simulink model "EV6_LUT_FourWheel_EV6Battery77p4kWh_PowerCorrected"  (R2024a)
settings: Solver=ode4  StartTime=0  StopTime=60  FixedStep=0.001  RelTol=1e-3
PreLoadFcn:
  | VSS_BICYCLE=Simulink.Variant('Dual=0');
  | VSS_DUAL=Simulink.Variant('Dual=1');
  | Dual=1;
  | load('DriveCycle2.mat')
PostLoadFcn:
  | if any(exist('dsrtsu_mdlpostloadfcn', 'file') ~= 0), dsrtsu_mdlpostloadfcn('Execute', bdroot); end
InitFcn:
  | , if any(exist('rtifpga_mdlclblib', 'file') ~= 0), rtifpga_mdlclblib('Init', bdroot); end,
  | , if any(exist('dsmpb_private', 'file') ~= 0), dsmpb_private('dsmpb_mdlclblib', 'Init', bdroot); end,
  | load('DriveCycle2.mat')
model workspace (MAT data in the model file):
  DiffRatio = 10.65
  EV6_2023_BattBranchCapacity_Ah = 55.5236728838
  EV6_2023_BattEnergy_kWh = 77.4
  EV6_2023_BattNominalVoltage_V = 697
  EV6_2023_BattNumCellsParallel = 2
  EV6_2023_BattNumCellsSeries = 192
  EV6_2023_BattOpenVoltCapBpts = [0 0.1 0.2 0.3 0.4 0.5 0.6 0.7 0.8 0.9 1]
  EV6_2023_BattOpenVoltTbl = [2.96762142548 3.40364281191 3.47417488548 3.54470541822 3.61523441014 3.68576186124 3.75628777151 3.82681214095 3.94527005036 4.07101207308 4.2120755254]
  EV6_2023_BattPackCapacity_Ah = 111.047345768
  EV6_2023_BattResistSocBpts = [0 0.2 0.4 0.6 0.8 1]
  EV6_2023_BattResistTbl = [0.0163620057716 0.0118174152018 0.00807187352333 0.00375663957972 0.00266904525531 0.00103635901355 0.0019014404175 0.0172368903217 0.0121226074867 0.00758541551769 0.00474065349228 0.00337561163613 ... (42 elements, 7x6)]
  EV6_2023_BattResistTempBpts = [243.1 253.1 263.1 273.1 283.1 298.1 313.1]
  EV6_2023_InitialPackOCV_V = 726.471714233
  EV6_2023_InitialSOC = 0.638878863672
  EV6_BattCellCapacity_Ah = 60.3
  EV6_BattInitialSOC = 0.638878863672
  EV6_BattOCV_Cell_V = [2.96762142548 3.40364281191 3.47417488548 3.54470541822 3.61523441014 3.68576186124 3.75628777151 3.82681214095 3.94527005036 4.07101207308 4.2120755254]
  EV6_BattOCV_SOC = [0 0.1 0.2 0.3 0.4 0.5 0.6 0.7 0.8 0.9 1]
  EV6_BattPackCapacity_Ah = 120.6
  EV6_BattParallelCells = 2
  EV6_BattResistanceSOC = [0 0.2 0.4 0.6 0.8 1]
  EV6_BattResistanceTable_Ohm = [0.0163620057716 0.0118174152018 0.00807187352333 0.00375663957972 0.00266904525531 0.00103635901355 0.0019014404175 0.0172368903217 0.0121226074867 0.00758541551769 0.00474065349228 0.00337561163613 ... (42 elements, 7x6)]
  EV6_BattResistanceTemp_K = [243.1 253.1 263.1 273.1 283.1 298.1 313.1]
  EV6_BattSeriesCells = 192
  EV6_FinalDriveRatio = 10.65
  EV6_TargetPackResistance_Ohm = 0.132763804608
  Gas = 0.383333333333
undefined symbols (not defined in the file): accel_bp_mps2, AccelCmd, ActTqLF_Nm_, ActTqLR_Nm_, ActTqRF_Nm_, ActTqRR_Nm_, BattChargeLimitMaxPwr, BattChargeLimitSocBpts, BattChargeLimitTbl, BattDischargeLimitSocBpts, BattDischargeLimitTbl, BattDischargeMaxPwr, BrakeMaxPrs, BrakeMaxTrq, ChassisDistCg2FrontAxle, ChassisDistCg2RearAxle, ChassisVehMass, CltchCmd, CoastDown, DecelCmd, DiscIntNeverNeededParam, EnvGravCnst, EnvPrs, EnvTemp, EV6_RegenTorqueGain, EV6_TractionTorqueGain, front_share_regen_3d, front_share_traction_3d, FuelSpecificGrav, GearCmd, h, InitStates, lgSw, limitedMCT, MCT, MtrEffSpdBpts, MtrEffTbl, MtrEffTrqBpts, MtrPwrMax, MtrTrqMax, out_1, pMCT, RealSimPara, Ref_speed, Ref_time, regen_torque_bp_Nm, speed_bp_kph, SteeringCmd, SupvsryCtrlRegenBrkCutOffTbl, SupvsryCtrlRegenSpdBpts, TestScnrioCycleNum, traction_torque_bp_Nm, US06, VEH
libraries: VSIGenLib x65, simulink x54, etargetslib x38, dsmpblib x24, vehdynlibtire x12, autolibshared x11, vehdynlibsuspension x7, vehdynlibtirecommon x7, autolibpowerinfoutils x6, autolibutils x5, autolibsharedcoupling x4, autolibmappedmotor x4
(part 7 of 19)

== system EV6_LUT_FourWheel_EV6Battery77p4kWh_PowerCorrected/Vehicle Under Test1/Vehicle/Rototest and ORNL Interface/RotoTrqPreprocess ==
  AxleTrqRaw : Inport
  Bus Selector1 : BusSelector  OutputSignals=ActTqLF_Nm_,ActTqRF_Nm_,ActTqLR_Nm_,ActTqRR_Nm_
  Compare To Constant : simulink/Logic and Bit Operations/Compare To Constant  relop=>=  const=-15  OutDataTypeStr=boolean
  Compare To Constant1 : simulink/Logic and Bit Operations/Compare To Constant  relop=<=  const=0  OutDataTypeStr=boolean
  Data Type Conversion{1..4} (4 alike) : DataTypeConversion  OutDataTypeStr=double  SaturateOnIntegerOverflow=off  RndMeth=Floor
  FirstOrderFilterTau{,1..3} (4 alike) : VSIGenLib/FirstOrderFilterTau  SystemSampleTime=-1  VariantActivationTime=update diagram  AllowFlexibleInterface=on  Latency=0  AutoFrameSizeCalculation=off
  Ground : Ground
  Logical Operator : Logic  AllPortsSameDT=off  OutDataTypeStr=boolean
  ManualTrq_Nm : Constant  Value=0
  Mux : Mux
  Mux1 : Mux
  SatTrq : Saturate  UpperLimit=1000  LowerLimit=-1000
  Tau : Constant  Value=0.01
  TorqueIn : Switch  Criteria=u2 > Threshold  SaturateOnIntegerOverflow=off  InputSameDT=off
  "TorqueIn " : Switch  Criteria=u2 > Threshold  SaturateOnIntegerOverflow=off  InputSameDT=off
  AxleTrqRoto : Outport
  AxleTrqVeh : Outport  Port=2
  wires:
  Data Type Conversion1/1 -> Mux/1  "LF"
  FirstOrderFilterTau2/1 -> Data Type Conversion3/1
  SatTrq/1 -> Compare To Constant/1, Compare To Constant1/1, "TorqueIn "/3
  Compare To Constant1/1 -> Logical Operator/2
  Bus Selector1/1 -> FirstOrderFilterTau/1  "<ActTqLF_Nm_>"
  FirstOrderFilterTau3/1 -> Data Type Conversion4/1
  FirstOrderFilterTau/1 -> Data Type Conversion1/1
  AxleTrqRaw/1 -> Bus Selector1/1
  Data Type Conversion2/1 -> Mux/2  "RF"
  FirstOrderFilterTau1/1 -> Data Type Conversion2/1
  "TorqueIn "/1 -> AxleTrqVeh/1  "Trq"
  TorqueIn/1 -> SatTrq/1
  Bus Selector1/2 -> FirstOrderFilterTau1/1  "<ActTqRF_Nm_>"
  Bus Selector1/3 -> FirstOrderFilterTau2/1  "<ActTqLR_Nm_>"
  Compare To Constant/1 -> Logical Operator/1
  Bus Selector1/4 -> FirstOrderFilterTau3/1  "<ActTqRR_Nm_>"
  [Switch] -> TorqueIn/2
  Mux1/1 -> TorqueIn/3
  Data Type Conversion3/1 -> Mux/3  "LR"
  Data Type Conversion4/1 -> Mux/4  "RR"
  Logical Operator/1 -> "TorqueIn "/2
  Ground/1 -> "TorqueIn "/1
  Tau/1 -> FirstOrderFilterTau3/2, FirstOrderFilterTau2/2, FirstOrderFilterTau1/2, FirstOrderFilterTau/2
  ManualTrq_Nm/1 -> Mux1/1, Mux1/2, Mux1/3, Mux1/4
  Mux/1 -> TorqueIn/1, AxleTrqRoto/1

== system EV6_LUT_FourWheel_EV6Battery77p4kWh_PowerCorrected/Vehicle Under Test1/Vehicle/Rototest and ORNL Interface/Subsystem2 ==
  AxlTorq : Inport
  BusCreator1 : BusCreator  Inputs=16
  BusCreator2 : BusCreator  Inputs=16
  Constant : Constant  Value=0
  Constant1 : Constant  Value=0
  Demux : Demux  Outputs=16
      settings: DisplayOption=none
  Terminator : Terminator
  Zero1 : Constant  Value=0
  Zero2 : Constant  Value=0
  Zero5 : Constant  Value=0
  BrakeUpd : Outport
  wires:
  AxlTorq/1 -> Terminator/1
  Demux/12 -> BusCreator1/12  "Brake IF Trq_Reg_trg RR"
  Zero5/1 -> BusCreator2/5, BusCreator2/6, BusCreator2/7, BusCreator2/8  "Brake IF Trq_PB RR"
  Demux/7 -> BusCreator1/7  "Brake IF Trq_PB RL"
  Demux/5 -> BusCreator1/5  "Brake IF Trq_PB FL"
  Demux/13 -> BusCreator1/13  "Brake IF Trq_DriveSrc_trg d0"
  BusCreator2/1 -> Demux/1
  Demux/10 -> BusCreator1/10  "Brake IF Trq_Reg_trg FR"
  Demux/8 -> BusCreator1/8  "Brake IF Trq_PB RR"
  Demux/1 -> BusCreator1/1  "Brake IF Trq_WB FL"
  BusCreator1/1 -> BrakeUpd/1
  Constant/1 -> BusCreator2/3, BusCreator2/4  "Brake IF Trq_WB RL"
  Demux/3 -> BusCreator1/3  "Brake IF Trq_WB RL"
  Demux/4 -> BusCreator1/4  "Brake IF Trq_WB RR"
  Zero1/1 -> BusCreator2/9, BusCreator2/10, BusCreator2/11, BusCreator2/12  "Brake IF Trq_Reg_trg RR"
  Demux/16 -> BusCreator1/16  "Brake IF Trq_DriveSrc_trg d3"
  Demux/2 -> BusCreator1/2  "Brake IF Trq_WB FR"
  Demux/15 -> BusCreator1/15  "Brake IF Trq_DriveSrc_trg d2"
  Demux/11 -> BusCreator1/11  "Brake IF Trq_Reg_trg RL"
  Zero2/1 -> BusCreator2/13, BusCreator2/14, BusCreator2/15, BusCreator2/16  "Brake IF Trq_DriveSrc_trg d3"
  Demux/14 -> BusCreator1/14  "Brake IF Trq_DriveSrc_trg d1"
  Constant1/1 -> BusCreator2/2, BusCreator2/1  "Brake IF Trq_WB FL"
  Demux/6 -> BusCreator1/6  "Brake IF Trq_PB FR"
  Demux/9 -> BusCreator1/9  "Brake IF Trq_Reg_trg FL"

== system EV6_LUT_FourWheel_EV6Battery77p4kWh_PowerCorrected/Vehicle Under Test1/Vehicle/Rototest and ORNL Interface/To Rototest with Band-Aid ==
  note: Switch = 0 Overides
      | Switch = 1 Model
  note: OutMode = 0 is Torque
      | OutMode = 1 is Speed
  note: Torque Model: Low speed
      | Speed Model: Normal speed
  SpeedCmd_rps : Inport
  AxleTrq_roto_Nm : Inport  Port=2
  BRAKE_PRESSED : Inport  Port=3
  Vehicle_Speed_kph : Inport  Port=4
  Band-Aid : Subsystem
  Demux : Demux
  Demux1 : Demux
  Demux2 : Demux
  Logging : Subsystem  Commented=on
  MasterSw : Constant  Value=0
  Mode Override : Subsystem
  ModeOut : Switch  Criteria=u2 > Threshold  SaturateOnIntegerOverflow=off  InputSameDT=off
  ModeSwitch : MultiPortSwitch  DataPortOrder=Zero-based contiguous  Inputs=2  zeroidx=on  SaturateOnIntegerOverflow=off  InputSameDT=off
  Mux2 : Mux
  Mux4 : Mux
  Mux5 : Mux
  RateLimSpd : RateLimiter  RisingSlewLimit=500  FallingSlewLimit=-500  SampleTimeMode=inherited
  RotoTestEthTx : Subsystem  AncestorBlock=VSIGenLib/RotoTestEthTx
      mask Display:
      | color('white')
      | disp('RotTestEthTx')
      | port_label('input', 1, 'RefLF_NmORrpm')
      | port_label('input', 2, 'RefRF_NmORrpm')
      | port_label('input', 3, 'RefLR_NmORrpm')
      | port_label('input', 4, 'RefRR_NmORrpm')
      | port_label('input', 5, 'SqTrRR')
      | port_label('input', 6, 'SqTrLR')
      | port_label('input', 7, 'SqTrRF')
      | port_label('input', 8, 'SqTrLF')
      | port_label('input', 9, 'SystemActive')
      | port_label('output', 1, 'Status (bool)')
      | port_label('output', 2, 'Sent Bytes (int)')
  SatSpd : Saturate  UpperLimit=500  LowerLimit=0
  Scope : Scope
  SpeedOut : Switch  Criteria=u2 > Threshold  SaturateOnIntegerOverflow=off  InputSameDT=off
  SystemActive : Constant  Value=0  OutDataTypeStr=uint8
  Transfer Fcn{,1..3} (4 alike) : TransferFcn  Denominator=[0.02 1]
  TrqSpd Override : Subsystem
  ZeroTorque : Constant  Value=0  OutDataTypeStr=uint8
  rads2rpm : Gain  Gain=9.5492965964254
  Out1 : Outport
  tag scope: Switch=global
  wires:
  Transfer Fcn3/1 -> RotoTestEthTx/4(RefRR_NmORrpm)
  Transfer Fcn2/1 -> RotoTestEthTx/3(RefLR_NmORrpm)
  Transfer Fcn1/1 -> RotoTestEthTx/2(RefRF_NmORrpm)
  Transfer Fcn/1 -> RotoTestEthTx/1(RefLF_NmORrpm)
  Vehicle_Speed_kph/1 -> Band-Aid/4(VehSpd_kph)
  BRAKE_PRESSED/1 -> Band-Aid/3(BRAKE_PRESSED)
  Band-Aid/2(OutSpd_rpm) -> SpeedOut/1
  Mux2/1 -> Band-Aid/1(InSpd_rpm)
  AxleTrq_roto_Nm/1 -> Band-Aid/2(InTrq_Nm)
  Mode Override/1(Ovr) -> ModeOut/3
  SpeedCmd_rps/1 -> rads2rpm/1
  Demux2/4 -> RotoTestEthTx/8(SpTqLF)
  Demux1/2 -> Transfer Fcn1/1
  Demux1/1 -> Transfer Fcn/1
  RotoTestEthTx/1(Output) -> Out1/1  "ByteSend"
  SystemActive/1 -> RotoTestEthTx/9(SystemActive)
  Demux2/2 -> RotoTestEthTx/6(SpTqLR)
  Demux2/3 -> RotoTestEthTx/7(SpTqRF)
  Demux1/3 -> Transfer Fcn2/1
  Demux2/1 -> RotoTestEthTx/5(SpTqRR)
  Mux5/1 -> ModeOut/1
  [Switch] -> ModeOut/2
  SatSpd/1 -> ModeSwitch/3  "Spd"
  [Switch] -> SpeedOut/2
  ModeOut/1 -> Demux2/1
  Band-Aid/1(OutMode) -> ModeSwitch/1, Mux5/1, Mux5/2, Mux5/3, Mux5/4
  Demux/4 -> Mux2/4  "RRIn"
  ModeSwitch/1 -> Demux1/1, Scope/1
  rads2rpm/1 -> Demux/1
  RateLimSpd/1 -> SatSpd/1
  SpeedOut/1 -> RateLimSpd/1
  Demux/1 -> Mux2/1  "LFIn"
  ZeroTorque/1 -> Mux4/1, Mux4/4, Mux4/3, Mux4/2
  TrqSpd Override/1(Ovr) -> SpeedOut/3
  MasterSw/1 -> [Switch]
  Demux/2 -> Mux2/2  "RFIn"
  Demux1/4 -> Transfer Fcn3/1
  Demux/3 -> Mux2/3  "LRIn"
  Mux4/1 -> ModeSwitch/2

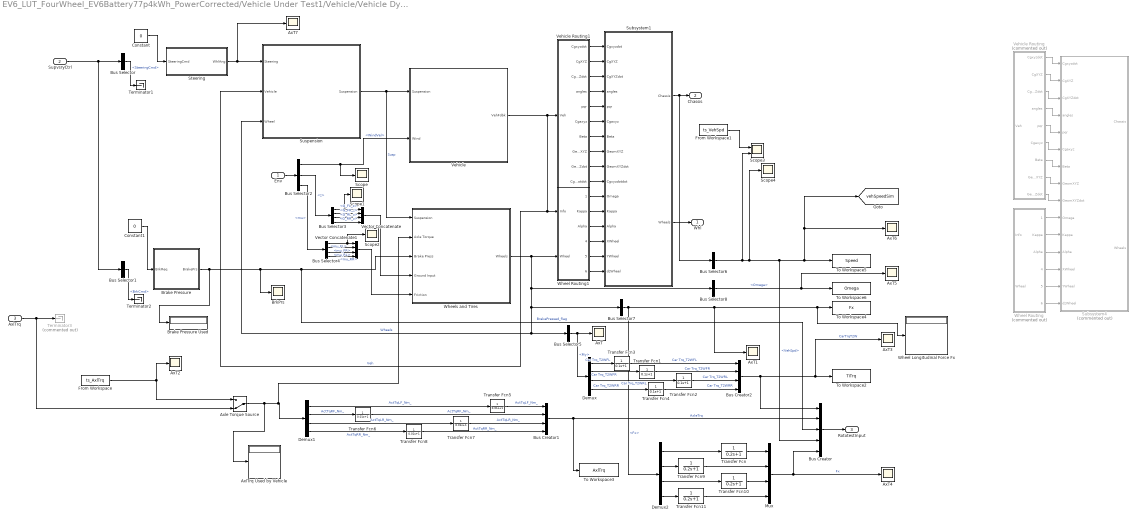
== system EV6_LUT_FourWheel_EV6Battery77p4kWh_PowerCorrected/Vehicle Under Test1/Vehicle/Vehicle Dynamics/Vehicle 14DOF ==
  Env : Inport
  SupvsryCtrl : Inport  Port=2
  AxlTrq : Inport  Port=3
  AxT{,1..7} (8 alike) : Scope
  AxlTrq Used by Vehicle : Display
  Axle Torque Source : ManualSwitch  CurrentSetting=0
  Brake Pressure : Subsystem
  Brake Pressure Used : Display
  BrkPrs : Scope
  Bus Creator : BusCreator  Inputs=5
  Bus Creator1 : BusCreator  Inputs=ActTqLF_Nm_,ActTqRF_Nm_,ActTqLR_Nm_,ActTqRR_Nm_
  Bus Creator2 : BusCreator  Inputs=Car Trq_T2WFL,Car Trq_T2WFR,Car Trq_T2WRL,Car Trq_T2WRR
  Bus Selector : BusSelector  OutputSignals=SteeringCmd
  Bus Selector1 : BusSelector  OutputSignals=BrkCmd
  Bus Selector2 : BusSelector  OutputSignals=WindVel,GndBus.z,GndBus.mu
  Bus Selector3 : BusSelector  OutputSignals=G_FL_z,G_FR_z,G_RL_z,G_RR_z
  Bus Selector4 : BusSelector  OutputSignals=mu_FL,mu_FR,mu_RL,mu_RR
  Bus Selector5 : BusSelector  OutputSignals=TireFrame.My
  Bus Selector6 : BusSelector  OutputSignals=VehSpd
  Bus Selector7 : BusSelector  OutputSignals=TireFrame.Fx
  Bus Selector8 : BusSelector  OutputSignals=TireFrame.Omega
  Constant : Constant  Value=0
  Constant1 : Constant  Value=0
  Demux : Demux
  Demux1 : Demux
  Demux2 : Demux
  From Workspace : FromWorkspace  VariableName=ts_AxlTrq
  From Workspace1 : FromWorkspace  VariableName=ts_VehSpd
  Mux : Mux
  Scope{,1..2,4} (4 alike) : Scope
  Scope3 : Scope  NumInputPorts=2
  Steering : Subsystem
  Subsystem1 : Subsystem
  Subsystem4 : Subsystem  Commented=on
  Suspension : Subsystem  Variant=on  VariantControlMode=label  LabelModeActiveChoice=3
      mask Display:
      | switch str2num(get_param(gcb,'ActiveVariant'))
      |     case 1
      |         image('suspdw.png');
      |     case 2
      |         image([imread('suspindmap.png');imread('suspsamap.png')]);
      |     case 3
      |          image([imread('suspmacp.png');imread('suspsacoil.png')]);
      |     case 4
      |          image('suspmacp.png');
      |     case 5
      |          image('suspindmap.png');
      | end
  Terminator1 : Terminator
  Terminator2 : Terminator
  Terminator3 : Terminator  Commented=on
  To Workspace2 : ToWorkspace  VariableName=TiTrq  SampleTime=-1
      settings: Save2DSignal=2-D array (concatenate along first dimension)
  To Workspace3 : ToWorkspace  VariableName=AxlTrq  SampleTime=-1
      settings: Save2DSignal=2-D array (concatenate along first dimension)
  To Workspace4 : ToWorkspace  VariableName=Fx  SampleTime=-1
      settings: Save2DSignal=2-D array (concatenate along first dimension)
  To Workspace5 : ToWorkspace  VariableName=Speed  SampleTime=-1
      settings: Save2DSignal=2-D array (concatenate along first dimension)
  To Workspace6 : ToWorkspace  VariableName=Omega  SampleTime=-1
      settings: Save2DSignal=2-D array (concatenate along first dimension)
  Transfer Fcn{,9..11} (4 alike) : TransferFcn  Denominator=[0.2 1]
  Transfer Fcn{1..4} (4 alike) : TransferFcn  Denominator=[0.1 1]
  Transfer Fcn{5..8} (4 alike) : TransferFcn  Denominator=[0.01 1]
  Vector Concatenate : Concatenate  NumInputs=4
  Vector Concatenate1 : Concatenate  NumInputs=4
  Vehicle : Subsystem
      mask Display: image('6dofcar.png');
  Vehicle Routing : Subsystem  Commented=on
  Vehicle Routing1 : Subsystem
  Wheel Longitudinal Force Fx : Display
  Wheel Routing : Subsystem  Commented=on
  Wheel Routing1 : Subsystem
  Wheels and Tires : Subsystem
      mask Display: image('wheel3dof.png')
  Whl : Outport
  Chassis : Outport  Port=2
  RototestInput : Outport  Port=3
  tag scope: vehSpeedSim=global
  wires:
  Vehicle Routing1/9(GeomXYZdot) -> Subsystem1/9(GeomXYZdot)
  Vehicle Routing1/8(GeomXYZ) -> Subsystem1/8(GeomXYZ)
  Vehicle Routing1/1(Cgxyzdot) -> Subsystem1/1(Cgxyzdot)
  Vehicle Routing1/5(pqr) -> Subsystem1/5(pqr)
  Vehicle Routing1/4(angles) -> Subsystem1/4(angles)
  Vehicle Routing1/3(CgXYZdot) -> Subsystem1/3(CgXYZdot)
  Vehicle Routing1/7(Beta) -> Subsystem1/7(Beta)
  Vehicle Routing1/2(CgXYZ) -> Subsystem1/2(CgXYZ)
  Vehicle Routing1/6(Cgaxyz) -> Subsystem1/6(Cgaxyz)
  Wheel Routing1/1(Omega) -> Subsystem1/11(Omega)
  Wheel Routing1/3(Alpha) -> Subsystem1/13(Alpha)
  Wheel Routing1/4(XWheel) -> Subsystem1/14(XWheel)
  Wheel Routing1/2(Kappa) -> Subsystem1/12(Kappa)
  Wheel Routing1/5(YWheel) -> Subsystem1/15(YWheel)
  Wheel Routing1/6(ZWheel) -> Subsystem1/16(dzWheel)
  Vehicle Routing1/10(Cgxyzdotdot) -> Subsystem1/10(Cgxyzdotdot)
  Vehicle Routing/8(GeomXYZ) -> Subsystem4/8(GeomXYZ)
  Vehicle Routing/6(Cgaxyz) -> Subsystem4/6(Cgaxyz)
  Vehicle Routing/3(CgXYZdot) -> Subsystem4/3(CgXYZdot)
  Vehicle Routing/9(GeomXYZdot) -> Subsystem4/9(GeomXYZdot)
  Vehicle Routing/4(angles) -> Subsystem4/4(angles)
  Vehicle Routing/7(Beta) -> Subsystem4/7(Beta)
  Wheel Routing/4(XWheel) -> Subsystem4/13(XWheel)
  Wheel Routing/1(Omega) -> Subsystem4/10(Omega)
  Wheel Routing/3(Alpha) -> Subsystem4/12(Alpha)
  Wheel Routing/5(YWheel) -> Subsystem4/14(YWheel)
  Wheel Routing/6(ZWheel) -> Subsystem4/15(dzWheel)
  Wheel Routing/2(Kappa) -> Subsystem4/11(Kappa)
  Vehicle Routing/1(Cgxyzdot) -> Subsystem4/1(Cgxyzdot)
  Vehicle Routing/5(pqr) -> Subsystem4/5(pqr)
  Vehicle Routing/2(CgXYZ) -> Subsystem4/2(CgXYZ)
  Transfer Fcn2/1 -> Bus Creator2/3  "Car Trq_T2WRL"
  Transfer Fcn4/1 -> Bus Creator2/4  "Car Trq_T2WRR"
  Demux/4 -> Transfer Fcn4/1  "Car Trq_T2WRR"
  Demux/1 -> Transfer Fcn3/1  "Car Trq_T2WFL"
  Demux/2 -> Transfer Fcn1/1  "Car Trq_T2WFR"
  Transfer Fcn1/1 -> Bus Creator2/2  "Car Trq_T2WFR"
  Demux/3 -> Transfer Fcn2/1  "Car Trq_T2WRL"
  Transfer Fcn3/1 -> Bus Creator2/1  "Car Trq_T2WFL"
  Mux/1 -> AxT4/1, Bus Creator/5  "Fx"
  Transfer Fcn11/1 -> Mux/4
  Demux2/1 -> Transfer Fcn/1
  Transfer Fcn/1 -> Mux/1
  Demux2/4 -> Transfer Fcn11/1
  Transfer Fcn9/1 -> Mux/2
  Demux2/2 -> Transfer Fcn9/1
  Transfer Fcn10/1 -> Mux/3
  Demux2/3 -> Transfer Fcn10/1
  Demux1/4 -> Transfer Fcn8/1  "ActTqRR_Nm_"
  Transfer Fcn7/1 -> Bus Creator1/3  "ActTqLR_Nm_"
  Demux1/1 -> Transfer Fcn5/1  "ActTqLF_Nm_"
  Transfer Fcn6/1 -> Bus Creator1/2  "ActTqRF_Nm_"
  Demux1/2 -> Transfer Fcn6/1  "ActTqRF_Nm_"
  Transfer Fcn8/1 -> Bus Creator1/4  "ActTqRR_Nm_"
  Demux1/3 -> Transfer Fcn7/1  "ActTqLR_Nm_"
  Transfer Fcn5/1 -> Bus Creator1/1  "ActTqLF_Nm_"
  Bus Creator/1 -> RototestInput/1
  Bus Selector8/1 -> To Workspace6/1, AxT5/1  "<Omega>"
  Bus Selector7/1 -> Wheel Longitudinal Force Fx/1, To Workspace4/1, AxT1/1, Demux2/1  "<Fx>"
  Subsystem1/1(Chassis) -> Chassis/1, Bus Selector6/1
  Bus Selector5/1 -> AxT/1, Demux/1  "<My>"
  Bus Creator2/1 -> To Workspace2/1, AxT3/1, Bus Creator/1  "CarTrqT2W"
  Bus Creator1/1 -> Bus Creator/2, To Workspace3/1  "AxleTrq"
  Brake Pressure/1(BrakePrs) -> Brake Pressure Used/1, Wheels and Tires/3(Brake Press), Bus Creator/3, BrkPrs/1  "BrakePressed_flag"
  Bus Selector6/1 -> Scope3/2, Scope4/1, Bus Creator/4, To Workspace5/1, [vehSpeedSim], AxT6/1  "<VehSpd>"
  Vector Concatenate1/1 -> Wheels and Tires/5(Friction)
  Bus Selector4/1 -> Vector Concatenate1/1, Scope2/1  "<mu_FL>"
  Bus Selector4/2 -> Vector Concatenate1/2  "<mu_FR>"
  Bus Selector4/3 -> Vector Concatenate1/3  "<mu_RL>"
  Bus Selector2/3 -> Bus Selector4/1  "<mu>"
  Bus Selector4/4 -> Vector Concatenate1/4  "<mu_RR>"
  Vector Concatenate/1 -> Wheels and Tires/4(Ground Input)
  Bus Selector3/4 -> Vector Concatenate/4  "<G_RR_z>"
  Bus Selector3/3 -> Vector Concatenate/3  "<G_RL_z>"
  Bus Selector3/2 -> Vector Concatenate/2  "<G_FR_z>"
  Bus Selector3/1 -> Vector Concatenate/1, Scope1/1  "<G_FL_z>"
  Bus Selector2/2 -> Bus Selector3/1  "<z>"
  Subsystem1/2(Wheels) -> Whl/1
  Env/1 -> Bus Selector2/1
  SupvsryCtrl/1 -> Bus Selector1/1, Bus Selector/1
  Steering/1(WhlAng) -> Suspension/1(Steering), AxT7/1
  Bus Selector2/1 -> Vehicle/2(Wind), Scope/1  "<WindVel>"
  Suspension/1(Suspension) -> Wheels and Tires/1(Suspension), Vehicle/1(Suspension)  "Susp"
  Vehicle/1(VehFdbk) -> Suspension/2(Vehicle), Wheel Routing1/1(Info), Vehicle Routing1/1(Veh)  "Veh"
  Wheels and Tires/1(Wheels) -> Wheel Routing1/2(Wheel), Bus Selector8/1, Suspension/3(Wheel), Bus Selector5/1, Bus Selector7/1  "Wheels"
  From Workspace1/1 -> Scope3/1
  From Workspace/1 -> Axle Torque Source/1, AxT2/1
  AxlTrq/1 -> Axle Torque Source/2, Terminator3/1
  Bus Selector1/1 -> Terminator2/1  "<BrkCmd>"
  Constant1/1 -> Brake Pressure/1(BrkReq)
  Constant/1 -> Steering/1(SteeringCmd)
  Bus Selector/1 -> Terminator1/1  "<SteeringCmd>"
  Axle Torque Source/1 -> Wheels and Tires/2(Axle Torque), Demux1/1, AxlTrq Used by Vehicle/1

== system EV6_LUT_FourWheel_EV6Battery77p4kWh_PowerCorrected/Vehicle Under Test1/Vehicle/Vehicle Dynamics/Vehicle 7DOF ==
  Env : Inport
  SupvsryCtrl : Inport  Port=2
  AxlTrq : Inport  Port=3
  Brake Pressure : Subsystem
  Bus Creator : BusCreator  Inputs=5
  Bus Selector : BusSelector  OutputSignals=SteeringCmd
  Bus Selector1 : BusSelector  OutputSignals=BrkCmd
  Bus Selector10 : BusSelector  OutputSignals=InertFrm.Geom.Disp.X,InertFrm.Geom.Disp.Y,InertFrm.Geom.Disp.Z  OutputAsBus=on
  Bus Selector11 : BusSelector  OutputSignals=InertFrm.Geom.Vel.Xdot,InertFrm.Geom.Vel.Ydot,InertFrm.Geom.Vel.Zdot  OutputAsBus=on
  Bus Selector12 : BusSelector  OutputSignals=BdyFrm.Geom.Ang.Beta
  Bus Selector13 : BusSelector  OutputSignals=BdyFrm.Cg.Vel.xdot,BdyFrm.Cg.Vel.ydot,BdyFrm.Cg.Vel.zdot  OutputAsBus=on
  Bus Selector2 : BusSelector  OutputSignals=WindVel,GndBus.z,GndBus.mu
  Bus Selector3 : BusSelector  OutputSignals=G_FL_z,G_FR_z,G_RL_z,G_RR_z
  Bus Selector4 : BusSelector  OutputSignals=mu_FL,mu_FR,mu_RL,mu_RR
  Bus Selector5 : BusSelector  OutputSignals=InertFrm.Cg.Disp.X,InertFrm.Cg.Disp.Y,InertFrm.Cg.Disp.Z  OutputAsBus=on
  Bus Selector6 : BusSelector  OutputSignals=InertFrm.Cg.Vel.Xdot,InertFrm.Cg.Vel.Ydot,InertFrm.Cg.Vel.Zdot  OutputAsBus=on
  Bus Selector7 : BusSelector  OutputSignals=BdyFrm.Cg.Acc.ax,BdyFrm.Cg.Acc.ay,BdyFrm.Cg.Acc.az  OutputAsBus=on
  Bus Selector8 : BusSelector  OutputSignals=InertFrm.Cg.Ang.phi,InertFrm.Cg.Ang.theta,InertFrm.Cg.Ang.psi  OutputAsBus=on
  Bus Selector9 : BusSelector  OutputSignals=BdyFrm.Cg.AngVel.p,BdyFrm.Cg.AngVel.q,BdyFrm.Cg.AngVel.r  OutputAsBus=on
  Bus to Vector{,1..7} (8 alike) : BusToVector
  Constant : Constant  Value=0
  For 3D Visualization : MATLAB Function  TreatAsAtomicUnit=on  mask{trackW=1.9, wheelB=ChassisDistCg2FrontAxle+ChassisDistCg2RearAxle}
      mask prompts: trackW "Vehicle track width, trackW [m]:"; wheelB "Vehicle wheelbase, wheelB [m]:"
      mask help: This block converts wheel ground height information into estimates of vehicle pitch, roll angles and vertical height in order to help in the visualization 3DOF based simulations with changes in terrain. Note that the resulting signals are only used as a visualization aid and do not account for the physical affects of the vehicle interacting with variable terrain or changes in orientation.
  Longitudinal Wheels 4DOF : Subsystem  VariantControl=1
      settings: AttributesFormatString=%<wheelMode>
  RototestDummy : Subsystem
  Steering : Subsystem
  Subsystem4 : Subsystem
  Terminator : Terminator
  Vector Concatenate : Concatenate  NumInputs=4
  Vector Concatenate1 : Concatenate  NumInputs=4
  Vector Concatenate2 : Concatenate  NumInputs=4
  Vehicle Body 3DOF External Longitudinal Wheels : Subsystem  Variant=on  VariantControlMode=label  VariantControl=Variant1  LabelModeActiveChoice=1
      settings: AttributesFormatString=%<trackMode>
  Whl : Outport
  Chassis : Outport  Port=2
  RototestInput : Outport  Port=3
  wires:
  RototestDummy/5(<Fx>) -> Bus Creator/5
  RototestDummy/4(<VehSpd>) -> Bus Creator/4
  RototestDummy/3(BrakePressed_flag) -> Bus Creator/3
  RototestDummy/2(AxleTrq) -> Bus Creator/2
  RototestDummy/1(CarTrqT2W) -> Bus Creator/1
  Bus Creator/1 -> RototestInput/1
  Longitudinal Wheels 4DOF/3(Omega) -> Subsystem4/10(Omega)  "Omega"
  Bus Selector7/1 -> Bus to Vector2/1
  Longitudinal Wheels 4DOF/6(zAxle) -> Subsystem4/15(dzWheel)  "dzWheel"
  Steering/1(WhlAng) -> Vehicle Body 3DOF External Longitudinal Wheels/1(WhlAng), Longitudinal Wheels 4DOF/1(WhlAng)
  Longitudinal Wheels 4DOF/4(Kappa) -> Subsystem4/11(Kappa)  "Kappa"
  Vehicle Body 3DOF External Longitudinal Wheels/2(" XWheel") -> Subsystem4/13(XWheel)  "XWheel"
  Brake Pressure/1(BrakePrs) -> Longitudinal Wheels 4DOF/3(BrkPrs)
  Bus Selector6/1 -> Bus to Vector1/1
  Vector Concatenate1/1 -> [mu], Longitudinal Wheels 4DOF/5(lam_mu)
  Longitudinal Wheels 4DOF/5(Alpha) -> Subsystem4/12(Alpha)  "Alpha"
  Bus to Vector3/1 -> For 3D Visualization/1(angleIn)
  Bus to Vector1/1 -> Subsystem4/3(CgXYZdot)  "CgXYZdot"
  [Ground] -> For 3D Visualization/3(GroundZ)
  Vehicle Body 3DOF External Longitudinal Wheels/1(" Info") -> Bus Selector5/1, Bus Selector6/1, Bus Selector9/1, Bus Selector7/1, Bus Selector12/1, Bus Selector8/1, Longitudinal Wheels 4DOF/6(VehFdbk), Bus Selector10/1, Bus Selector11/1, Bus Selector13/1
  AxlTrq/1 -> Longitudinal Wheels 4DOF/2(AxlTrq)
  Bus to Vector/1 -> Subsystem4/2(CgXYZ)  "CgXYZ"
  Vector Concatenate/1 -> [Ground], Longitudinal Wheels 4DOF/4(Gnd)
  Vehicle Body 3DOF External Longitudinal Wheels/3(" YWheel") -> Subsystem4/14(YWheel)  "YWheel"
  Bus to Vector4/1 -> Subsystem4/5(pqr)  "pqr"
  Longitudinal Wheels 4DOF/2(RearAxlF) -> Vehicle Body 3DOF External Longitudinal Wheels/3("FwR ")
  [mu] -> Vehicle Body 3DOF External Longitudinal Wheels/5(Friction)
  Bus Selector9/1 -> Bus to Vector4/1
  Bus Selector11/1 -> Bus to Vector6/1
  Longitudinal Wheels 4DOF/1(FrntAxlF) -> Vehicle Body 3DOF External Longitudinal Wheels/2("FwF ")
  Bus Selector10/1 -> Bus to Vector5/1
  Bus to Vector7/1 -> Subsystem4/1(Cgxyzdot)  "Cgxyzdot"
  Bus Selector13/1 -> Bus to Vector7/1
  Bus to Vector6/1 -> Subsystem4/9(GeomXYZdot)  "GeomXYZdot"
  For 3D Visualization/2(GeomXYZ) -> Subsystem4/8(GeomXYZ)  "GeomXYZ"
  For 3D Visualization/1(angles) -> Subsystem4/4(angles)  "angles"
  Bus Selector5/1 -> Bus to Vector/1
  Bus Selector12/1 -> Subsystem4/7(Beta)  "<Beta>"
  Bus to Vector5/1 -> For 3D Visualization/2(GemoXYZIn)
  Bus Selector8/1 -> Bus to Vector3/1
  Bus to Vector2/1 -> Subsystem4/6(Cgaxyz)  "Cgaxyz"
  Constant/1 -> Vector Concatenate2/1, Vector Concatenate2/2, Vector Concatenate2/3, Vector Concatenate2/4
  Vector Concatenate2/1 -> Terminator/1
  Bus Selector4/1 -> Vector Concatenate1/1  "<mu_FL>"
  Bus Selector4/2 -> Vector Concatenate1/2  "<mu_FR>"
  Bus Selector4/3 -> Vector Concatenate1/3  "<mu_RL>"
  Bus Selector2/3 -> Bus Selector4/1  "<mu>"
  Bus Selector4/4 -> Vector Concatenate1/4  "<mu_RR>"
  Bus Selector3/4 -> Vector Concatenate/4  "<G_RR_z>"
  Bus Selector3/3 -> Vector Concatenate/3  "<G_RL_z>"
  Bus Selector3/2 -> Vector Concatenate/2  "<G_FR_z>"
  Bus Selector3/1 -> Vector Concatenate/1  "<G_FL_z>"
  Bus Selector2/2 -> Bus Selector3/1  "<z>"
  Subsystem4/1(Chassis) -> Chassis/1
  Subsystem4/2(Wheels) -> Whl/1
  Env/1 -> Bus Selector2/1
  Bus Selector1/1 -> Brake Pressure/1(BrkReq)  "<BrkCmd>"
  SupvsryCtrl/1 -> Bus Selector1/1, Bus Selector/1
  Bus Selector/1 -> Steering/1(SteeringCmd)  "<SteeringCmd>"
  Bus Selector2/1 -> Vehicle Body 3DOF External Longitudinal Wheels/4(WindXYZ)  "<WindVel>"

== system EV6_LUT_FourWheel_EV6Battery77p4kWh_PowerCorrected/Vehicle Under Test1/Vehicle/Vehicle Dynamics/Vehicle Longitudinal ==
  Env : Inport
  SupvsryCtrl : Inport  Port=2
  AxlTrq : Inport  Port=3
  Brake Pressure : Subsystem
  Bus Creator : BusCreator  Inputs=5
  Bus Selector1 : BusSelector  OutputSignals=BrkCmd
  Bus Selector2 : BusSelector  OutputSignals=RoadGrade,WindVel,GndBus.z,GndBus.mu
  Bus Selector3 : BusSelector  OutputSignals=G_FL_z,G_FR_z,G_RL_z,G_RR_z
  Bus Selector4 : BusSelector  OutputSignals=mu_FL,mu_FR,mu_RL,mu_RR
  Constant : Constant  Value=0
  Longitudinal Wheels : Subsystem  AncestorBlock=LibWheels/Longitudinal Wheels and Brakes
  RototestDummy : Subsystem
  Selector : Selector  InputPortWidth=3  IndexOptions=Index vector (dialog)  Indices=1  OutputSizes=1
  Terminator : Terminator
  Terminator1 : Terminator
  Vector Concatenate : Concatenate  NumInputs=4
  Vector Concatenate1 : Concatenate  NumInputs=4
  Vector Concatenate2 : Concatenate  NumInputs=4
  Vehicle Body : Subsystem
  Whl : Outport
  Chassis : Outport  Port=2
  RototestInput : Outport  Port=3
  wires:
  RototestDummy/1(CarTrqT2W) -> Bus Creator/1
  RototestDummy/2(AxleTrq) -> Bus Creator/2
  RototestDummy/3(BrakePressed_flag) -> Bus Creator/3
  RototestDummy/4(<VehSpd>) -> Bus Creator/4
  RototestDummy/5(<Fx>) -> Bus Creator/5
  Bus Creator/1 -> RototestInput/1
  Selector/1 -> Vehicle Body/2(WindX)
  Bus Selector2/1 -> Vehicle Body/1(RoadGrade)  "<RoadGrade>"
  Bus Selector2/2 -> Selector/1  "<WindVel>"
  AxlTrq/1 -> Longitudinal Wheels/2(AxleTorq)
  Bus Selector3/3 -> Vector Concatenate/3  "<G_RL_z>"
  Bus Selector1/1 -> Brake Pressure/1(BrkReq)  "<BrkCmd>"
  Bus Selector4/4 -> Vector Concatenate1/4  "<mu_RR>"
  Constant/1 -> Vector Concatenate2/1, Vector Concatenate2/2, Vector Concatenate2/3, Vector Concatenate2/4
  SupvsryCtrl/1 -> Bus Selector1/1
  Bus Selector3/2 -> Vector Concatenate/2  "<G_FR_z>"
  Bus Selector4/3 -> Vector Concatenate1/3  "<mu_RL>"
  Vector Concatenate/1 -> Terminator/1
  Env/1 -> Bus Selector2/1
  Bus Selector2/3 -> Bus Selector3/1  "<z>"
  Bus Selector3/4 -> Vector Concatenate/4  "<G_RR_z>"
  Bus Selector3/1 -> Vector Concatenate/1  "<G_FL_z>"
  Bus Selector4/2 -> Vector Concatenate1/2  "<mu_FR>"
  Brake Pressure/1(BrakePrs) -> Longitudinal Wheels/1(BrkPrs)
  Vector Concatenate1/1 -> Terminator1/1
  Bus Selector2/4 -> Bus Selector4/1  "<mu>"
  Bus Selector4/1 -> Vector Concatenate1/1  "<mu_FL>"
  Longitudinal Wheels/1(Whl) -> Whl/1
  Vehicle Body/1(Chassis) -> Chassis/1
  connections:
  Vehicle Body/LConn1 -- Longitudinal Wheels/RConn1
  Longitudinal Wheels/RConn2 -- Vehicle Body/LConn2

== system EV6_LUT_FourWheel_EV6Battery77p4kWh_PowerCorrected/Vehicle Under Test1/Vehicle/Actuation and Outputs/MOOG Brake Actuator/ CAN Settings ==
  " CAN diagnostic Counter" : Subsystem  Commented=on  mask{TimeOutDuration=0.1}
      mask prompts: TimeOutDuration "CAN Time Out Duration"
  Constant : Constant
  Data Type Conversion1 : DataTypeConversion  Commented=on  SaturateOnIntegerOverflow=off  RndMeth=Floor
  Data Type Conversion3 : DataTypeConversion  SaturateOnIntegerOverflow=off  RndMeth=Floor
  "RPDO3 Enable " : Constant
  RPDO3 period : Constant  Value=0.001
  RPDO3\PDU Features\PDU Cyclic Timing Control\RPDO3 Timing Control Period [BrakeAct_Config\Simulated ECUs\CANOpen_MOOG_02\Controller\TX\PDUs] : dsmpblib/Data Outport  Priority=-10000  Commented=on
      settings: SourceProductName=dSPACE Model Interface Package for Simulink (MIPS)
  RPDO3\PDU Features\PDU Enable\RPDO3 Enable [BrakeAct_Config\Simulated ECUs\CANOpen_MOOG_02\Controller\TX\PDUs] : dsmpblib/Data Outport  Priority=-10000  Commented=on
      settings: SourceProductName=dSPACE Model Interface Package for Simulink (MIPS)
  TPDO3\PDU Features\PDU RX Status\TPDO3 Counter [BrakeAct_Config\Simulated ECUs\CANOpen_MOOG_02\Controller\RX\PDUs] : dsmpblib/Data Inport  Priority=10000  Commented=on
      settings: SourceProductName=dSPACE Model Interface Package for Simulink (MIPS)
  Terminator : Terminator
  Terminator1 : Terminator
  CAN_CommsOK_Flg : Outport
  wires:
  Data Type Conversion1/1 -> " CAN diagnostic Counter"/1(RX Counter)
  TPDO3\PDU Features\PDU RX Status\TPDO3 Counter [BrakeAct_Config\Simulated ECUs\CANOpen_MOOG_02\Controller\RX\PDUs]/1 -> Data Type Conversion1/1
  RPDO3 period/1 -> Terminator1/1
  Data Type Conversion3/1 -> Terminator/1
  "RPDO3 Enable "/1 -> Data Type Conversion3/1
  Constant/1 -> CAN_CommsOK_Flg/1

== system EV6_LUT_FourWheel_EV6Battery77p4kWh_PowerCorrected/Vehicle Under Test1/Vehicle/Actuation and Outputs/MOOG Brake Actuator/MOOG Interface ==
  note: RAV4
      | Min an Max stops need adjusting otherwise:
      | - brake lights come on at 13% (with ajustment, it comes on at 2-3%
      | - 100% pedal can cause the actuator to generate a fault (maybe over current)
      | Min Offset +5500
      | Max Offset -5500
      |
      | Mach-e
      | Min Offset +5500
      | Max Offset -3500
      | this results in brake lights coming on at 4% and off at 1%
      |
      | total travel needs to be more than 35000 for valid range,
      | otherwise, brake booster was most likely not active
  CAN_CommsOK_Flg : Inport
  TargetPosition [pct] : Inport  Port=2
  StatusWord in : Inport  Port=3
  ActualPosition_cnt in : Inport  Port=4
  Mode of operation in : Inport  Port=5
  ActuatorMinTravelForReady : Constant  Value=35000
  Bus Creator : BusCreator  Inputs=2
  Constant1 : Constant  Value=100
  Constant2 : Constant  Value=100
  Data Type Conversion : DataTypeConversion  SaturateOnIntegerOverflow=off  RndMeth=Floor
  Data Type Conversion1 : DataTypeConversion  SaturateOnIntegerOverflow=off  RndMeth=Floor
  Display{2..5} (4 alike) : Display
  Gain : Gain
  Gain1 : Gain
  Gain2 : Gain
  MOOG State Machine : Stateflow chart  TreatAsAtomicUnit=on
  Max Stop Adjustment : Subsystem  TreatAsAtomicUnit=on
  Memory : Memory  InheritSampleTime=on
  Memory1 : Memory  InheritSampleTime=on
  Memory2 : Memory  InheritSampleTime=on
  Min Stop Adjustment : Subsystem  TreatAsAtomicUnit=on
  MoogResetCmd : Constant  Value=0
  PositionLearningTrigger : Constant  Value=0
  Product : Product  Inputs=*/*
  Product1 : Product  Inputs=*/*
  Rising edge : Subsystem
  Rising edge1 : Subsystem
  Sum : Sum  Inputs=|+-
  Sum1 : Sum  Inputs=|++
  Sum2 : Sum  Inputs=|+-
  Terminator1 : Terminator
  Commands : Outport
  ActualPosition [pct] : Outport  Port=2
  BrakeActuatorReady : Outport  Port=3
  wires:
  ActuatorMinTravelForReady/1 -> MOOG State Machine/7(ActuatorMinTravelForReady)
  CAN_CommsOK_Flg/1 -> MOOG State Machine/1(CAN_CommsOK_Flg)
  Memory2/1 -> Min Stop Adjustment/Enable, Max Stop Adjustment/Enable
  Memory1/1 -> Min Stop Adjustment/1(In1)
  Memory/1 -> Max Stop Adjustment/1(In1)
  [MinStop_cnt] -> Sum1/2
  Min Stop Adjustment/1(Out1) -> [MinStop_cnt]  "MinStop_cnt"
  Max Stop Adjustment/1(Out1) -> [MaxStop_cnt]  "MaxStop_cnt"
  Rising edge1/1(Out) -> MOOG State Machine/3(PositionLearningTrigger)
  PositionLearningTrigger/1 -> Rising edge1/1(In)
  Rising edge/1(Out) -> MOOG State Machine/2(ResetCmd)
  MoogResetCmd/1 -> Rising edge/1(In)
  Data Type Conversion1/1 -> MOOG State Machine/5(ActualPosition_cnt)  "ActualPosition_cnt"
  Gain2/1 -> Bus Creator/2  "TargetPositionFinal_cnt"
  MOOG State Machine/2(PositionCmd) -> Gain2/1
  MOOG State Machine/8(LearningComplete) -> Memory2/1  "LearningComplete"
  MOOG State Machine/9(MaxStop) -> Memory/1  "MaxStop"
  MOOG State Machine/10(MinStop) -> Memory1/1  "MinStop"
  MOOG State Machine/7(MoogOpMode) -> Display5/1  "MoogOpMode"
  MOOG State Machine/6(InitComplete) -> Display4/1  "InitComplete"
  MOOG State Machine/5(MoogSMState) -> Display3/1  "MoogSMState"
  Mode of operation in/1 -> Gain1/1
  ActualPosition_cnt in/1 -> Gain/1
  Data Type Conversion/1 -> MOOG State Machine/4(StatusWord)  "StatusWord"
  StatusWord in/1 -> Data Type Conversion/1
  Product1/1 -> ActualPosition [pct]/1  "ActualPosition_pct"
  Constant1/1 -> Product1/3
  Sum2/1 -> Product1/1
  [MinStop_cnt] -> Sum2/2
  Product/1 -> Sum1/1
  Gain1/1 -> Terminator1/1  "Mode of operation"
  Gain/1 -> Sum2/1, Data Type Conversion1/1
  Constant2/1 -> Product/2
  TargetPosition [pct]/1 -> Product/1  "TargetPosition_pct"
  Sum/1 -> Product/3, Product1/2
  MOOG State Machine/4(FaultCntr) -> Display2/1  "FaultCounter"
  MOOG State Machine/3(Actuator_Ready) -> BrakeActuatorReady/1  "Actuator_Ready"
  MOOG State Machine/1(ControlWord) -> Bus Creator/1  "ControlWord"
  [MinStop_cnt] -> Sum/2
  [MaxStop_cnt] -> Sum/1
  Bus Creator/1 -> Commands/1
  Sum1/1 -> MOOG State Machine/6(TargetPosition_cnt)  "TargetPosition_cnt"

== system EV6_LUT_FourWheel_EV6Battery77p4kWh_PowerCorrected/Vehicle Under Test1/Vehicle/Battery/Battery/EV6 Speed Mode Power Correction ==
  VehicleSpeed_mps : Inport
  FrontCurrent_A : Inport  Port=2
  RearCurrent_A : Inport  Port=3
  Base Current to Power : Gain  Gain=726.5/1000
  Base Motor Current Sum : Sum
  Low Power Correction LUT : Lookup_n-D  NumberOfTableDimensions=1  BreakpointsForDimension1=[1.25 3.75 6.25 8.75 11.25 13.75 17.5 22.5 27.5]  Table=[0.2676226994945869 0.1984316412329003 0.06004952470952702 0 0 0 0 0.0007805933368547949 0.0007805933368547949]  ExtrapMethod=Clip  InternalRulePriority=Speed  RndMeth=Simplest
  Negative Base Power : Gain  Gain=-1
  Power Correction to Current : Gain  Gain=1000/726.5
  Regen Correction LUT : Lookup_n-D  NumberOfTableDimensions=1  BreakpointsForDimension1=[1.25 3.75 6.25 8.75 11.25 13.75 17.5 22.5 27.5]  Table=[1.713948799890918 1.389238301395071 0.7038217909916348 -0.2403465168134532 -0.7851254419364538 -1.106337783241926 -1.05232617783835 -1.019658775252617 -0.7965172632084265]  ExtrapMethod=Clip  InternalRulePriority=Speed  RndMeth=Simplest
  Regen or Low Power : Switch  Criteria=u2 > Threshold  Threshold=0.5  SaturateOnIntegerOverflow=off  InputSameDT=off
  Traction Correction LUT : Lookup_n-D  NumberOfTableDimensions=1  BreakpointsForDimension1=[1.25 3.75 6.25 8.75 11.25 13.75 17.5 22.5 27.5]  Table=[0.4174562053869272 0.3686076794070289 0.2347220132221115 0.04999371281964825 -0.1523755981086843 -0.2710860131396209 -0.3476574654693272 -0.4175376171516637 -0.4812193851521126]  ExtrapMethod=Clip  InternalRulePriority=Speed  RndMeth=Simplest
  Traction or Other Mode : Switch  Criteria=u2 > Threshold  Threshold=0.5  SaturateOnIntegerOverflow=off  InputSameDT=off
  CorrectionCurrent_A : Outport
  CorrectionPower_kW : Outport  Port=2
  BasePower_kW : Outport  Port=3
  wires:
  VehicleSpeed_mps/1 -> Traction Correction LUT/1, Regen Correction LUT/1, Low Power Correction LUT/1
  FrontCurrent_A/1 -> Base Motor Current Sum/1
  RearCurrent_A/1 -> Base Motor Current Sum/2
  Base Motor Current Sum/1 -> Base Current to Power/1
  Base Current to Power/1 -> Negative Base Power/1, Traction or Other Mode/2, BasePower_kW/1
  Regen Correction LUT/1 -> Regen or Low Power/1
  Negative Base Power/1 -> Regen or Low Power/2
  Low Power Correction LUT/1 -> Regen or Low Power/3
  Traction Correction LUT/1 -> Traction or Other Mode/1
  Regen or Low Power/1 -> Traction or Other Mode/3
  Traction or Other Mode/1 -> Power Correction to Current/1, CorrectionPower_kW/1
  Power Correction to Current/1 -> CorrectionCurrent_A/1

== system EV6_LUT_FourWheel_EV6Battery77p4kWh_PowerCorrected/Vehicle Under Test1/Vehicle/Battery/Battery/Lithium Ion Battery Pack1 ==
  note: Info
  BattCurr : Inport  Unit=A
  BattTemp : Inport  Port=2  Unit=K
  Datasheet Battery Internal : Subsystem  AncestorBlock=autolibbatterycommon/Datasheet Battery Internal
  Info Bus : autolibbatterycommon/Info  RefBlkName='autolibdatasheetbattery/Datasheet Battery'
      settings: SourceProductName=Powertrain Blockset
  Output Passthrough : autolibbatterycommon/Output Passthrough  SystemSampleTime=-1  VariantActivationTime=update diagram  AllowFlexibleInterface=on  Latency=0  AutoFrameSizeCalculation=off
      settings: SourceProductName=Powertrain Blockset
  Info : Outport  VectorParamsAs1DForOutWhenUnconnected=off
  BattVolt : Outport  Port=2  Unit=V  VectorParamsAs1DForOutWhenUnconnected=off
  wires:
  [LdAmpHr] -> Info Bus/1
  [BattSoc] -> Info Bus/2
  Info Bus/1 -> Info/1
  BattCurr/1 -> Datasheet Battery Internal/1(BattCurr)
  BattTemp/1 -> Datasheet Battery Internal/2(BattTemp)
  Datasheet Battery Internal/4(BattSoc) -> [BattSoc]
  Datasheet Battery Internal/3(LdAmpHr) -> [LdAmpHr]
  Datasheet Battery Internal/2(OutVoltUnfilt) -> Output Passthrough/1
  Datasheet Battery Internal/5(BattPwrLoss) -> [BattPwrLoss]
  [LdCurrFeed] -> Info Bus/3
  Datasheet Battery Internal/1(LdCurrFeed) -> [LdCurrFeed]
  [BattVolt] -> Info Bus/4
  Output Passthrough/1 -> [BattVolt], BattVolt/1
  [BattPwrLoss] -> Info Bus/5

== system EV6_LUT_FourWheel_EV6Battery77p4kWh_PowerCorrected/Vehicle Under Test1/Vehicle/Driver and Drive Cycle/Driver and PI with FF Control/Speed controller set ==
  RefSpd [km/hr] : Inport
  VehSpd : Inport  Port=2
  Control selection : Constant
  In-house CAVE : Subsystem  VariantControl=varaint1
  Multiport Switch1 : MultiPortSwitch  SaturateOnIntegerOverflow=off  InputSameDT=off
  Multiport Switch2 : MultiPortSwitch  SaturateOnIntegerOverflow=off  InputSameDT=off
  Multiport Switch3 : MultiPortSwitch  SaturateOnIntegerOverflow=off  InputSameDT=off
  PIF : Subsystem  VariantControl=varaint2
  Predictive : Subsystem  VariantControl=varaint3
  Scope : Scope  NumInputPorts=2
  Speed tracking controller : Subsystem  Commented=on  Variant=on  VariantControlMode=label  VariantControl=Variant1  LabelModeActiveChoice=varaint1  PropagateVariantConditions=on
  AccelPedalCmd : Outport
  BrakePedalCmd : Outport  Port=2
  BrakeSwitch : Outport  Port=3
  wires:
  VehSpd/1 -> Scope/2, In-house CAVE/2(VehSpd), Predictive/2(VehSpd), PIF/2(VehSpd)
  Multiport Switch1/1 -> AccelPedalCmd/1  "AccelPedalCmd"
  Multiport Switch2/1 -> BrakePedalCmd/1  "BrakePedalCmd"
  Multiport Switch3/1 -> BrakeSwitch/1  "BrakeSwitch"
  Predictive/3(BrakeSwitch) -> Multiport Switch3/4
  PIF/3(BrakeSwitch) -> Multiport Switch3/3
  In-house CAVE/3(BrakeSwitch) -> Multiport Switch3/2
  Predictive/2(BrakePedalCmd) -> Multiport Switch2/4
  PIF/2(BrakePedalCmd) -> Multiport Switch2/3
  In-house CAVE/2(BrakePedalCmd) -> Multiport Switch2/2
  Predictive/1(AccelPedalCmd) -> Multiport Switch1/4
  PIF/1(AccelPedalCmd) -> Multiport Switch1/3
  In-house CAVE/1(AccelPedalCmd) -> Multiport Switch1/2
  RefSpd [km/hr]/1 -> Scope/1, PIF/1(RefSpd [km/hr]), Predictive/1(RefSpd [km/hr]), In-house CAVE/1(RefSpd [km/hr])
  Control selection/1 -> Multiport Switch1/1, Multiport Switch2/1, Multiport Switch3/1

== system EV6_LUT_FourWheel_EV6Battery77p4kWh_PowerCorrected/Vehicle Under Test1/Vehicle/Front Wheel Drive/Ideal Diff/Power Bus ==
  DriveshftTrq : Inport
  Speed : Inport  Port=2
  Bus Creator : BusCreator  Inputs=1
  Bus Creator5 : BusCreator  Inputs=2
  Bus Creator6 : BusCreator  Inputs=3
  Bus Creator7 : BusCreator  Inputs=1
  Constant : Constant  Value=0
  Constant1 : Constant  Value=0
  Constant2 : Constant  Value=0
  Demux : Demux  Outputs=3
  Power Accounting Bus Creator : autolibpowerinfoutils/Power Accounting Bus Creator  AssctBlkSelPopup=Parent reference block  RefBlkName='autolibshareddiff/Open Differential'  PwrTrnsfrdCheckBox=on  PwrNotTrnsfrdCheckBox=on  PwrStoredCheckBox=on  aMode=aMode
  Signal Specification5 : SignalSpecification  Unit=W
  Transferred Power : Product
  Vector Concatenate : Concatenate  NumInputs=3
  PwrInfo : Outport
  wires:
  Bus Creator/1 -> Power Accounting Bus Creator/1
  Power Accounting Bus Creator/1 -> PwrInfo/1  "PwrInfo"
  Bus Creator5/1 -> Power Accounting Bus Creator/2
  Bus Creator6/1 -> Bus Creator/1  "PwrTrnsfrd"
  Transferred Power/1 -> Signal Specification5/1
  Signal Specification5/1 -> Vector Concatenate/3, Vector Concatenate/2, Vector Concatenate/1  "PwrDriveshft"
  Constant/1 -> Bus Creator5/1  "PwrMechLoss"
  Demux/3 -> Bus Creator6/3  "PwrAxl2"
  DriveshftTrq/1 -> Transferred Power/1
  Bus Creator7/1 -> Power Accounting Bus Creator/3
  Demux/2 -> Bus Creator6/2  "PwrAxl1"
  Demux/1 -> Bus Creator6/1  "PwrDriveshft"
  Speed/1 -> Transferred Power/2
  Vector Concatenate/1 -> Demux/1
  Constant1/1 -> Bus Creator5/2  "PwrDampLoss"
  Constant2/1 -> Bus Creator7/1  "PwrStoredShft"

== system EV6_LUT_FourWheel_EV6Battery77p4kWh_PowerCorrected/Vehicle Under Test1/Vehicle/Front Wheel Drive/Ideal Diff AWD/Power Bus ==
  DriveshftTrq : Inport
  Speed : Inport  Port=2
  Bus Creator : BusCreator  Inputs=1
  Bus Creator5 : BusCreator  Inputs=2
  Bus Creator6 : BusCreator  Inputs=3
  Bus Creator7 : BusCreator  Inputs=1
  Constant : Constant  Value=0
  Constant1 : Constant  Value=0
  Constant2 : Constant  Value=0
  Demux : Demux  Outputs=3
  Power Accounting Bus Creator : autolibpowerinfoutils/Power Accounting Bus Creator  AssctBlkSelPopup=Parent reference block  RefBlkName='autolibshareddiff/Open Differential'  PwrTrnsfrdCheckBox=on  PwrNotTrnsfrdCheckBox=on  PwrStoredCheckBox=on  aMode=aMode
  Signal Specification5 : SignalSpecification  Unit=W
  Transferred Power : Product
  Vector Concatenate : Concatenate  NumInputs=3
  PwrInfo : Outport
  wires:
  Bus Creator/1 -> Power Accounting Bus Creator/1
  Power Accounting Bus Creator/1 -> PwrInfo/1  "PwrInfo"
  Bus Creator5/1 -> Power Accounting Bus Creator/2
  Bus Creator6/1 -> Bus Creator/1  "PwrTrnsfrd"
  Transferred Power/1 -> Signal Specification5/1
  Signal Specification5/1 -> Vector Concatenate/3, Vector Concatenate/2, Vector Concatenate/1  "PwrDriveshft"
  Constant/1 -> Bus Creator5/1  "PwrMechLoss"
  Demux/3 -> Bus Creator6/3  "PwrAxl2"
  DriveshftTrq/1 -> Transferred Power/1
  Bus Creator7/1 -> Power Accounting Bus Creator/3
  Demux/2 -> Bus Creator6/2  "PwrAxl1"
  Demux/1 -> Bus Creator6/1  "PwrDriveshft"
  Speed/1 -> Transferred Power/2
  Vector Concatenate/1 -> Demux/1
  Constant1/1 -> Bus Creator5/2  "PwrDampLoss"
  Constant2/1 -> Bus Creator7/1  "PwrStoredShft"

== system EV6_LUT_FourWheel_EV6Battery77p4kWh_PowerCorrected/Vehicle Under Test1/Vehicle/Front Wheel Drive/Real Diff/Power Bus ==
  DriveshftTrq : Inport
  Speed : Inport  Port=2
  Bus Creator : BusCreator  Inputs=1
  Bus Creator5 : BusCreator  Inputs=2
  Bus Creator6 : BusCreator  Inputs=3
  Bus Creator7 : BusCreator  Inputs=1
  Constant : Constant  Value=0
  Constant1 : Constant  Value=0
  Constant2 : Constant  Value=0
  Demux : Demux  Outputs=3
  Power Accounting Bus Creator : autolibpowerinfoutils/Power Accounting Bus Creator  AssctBlkSelPopup=Parent reference block  RefBlkName='autolibshareddiff/Open Differential'  PwrTrnsfrdCheckBox=on  PwrNotTrnsfrdCheckBox=on  PwrStoredCheckBox=on  aMode=aMode
  Signal Specification5 : SignalSpecification  Unit=W
  Transferred Power : Product
  Vector Concatenate : Concatenate  NumInputs=3
  PwrInfo : Outport
  wires:
  Bus Creator/1 -> Power Accounting Bus Creator/1
  Power Accounting Bus Creator/1 -> PwrInfo/1  "PwrInfo"
  Bus Creator5/1 -> Power Accounting Bus Creator/2
  Bus Creator6/1 -> Bus Creator/1  "PwrTrnsfrd"
  Transferred Power/1 -> Signal Specification5/1
  Signal Specification5/1 -> Vector Concatenate/3, Vector Concatenate/2, Vector Concatenate/1  "PwrDriveshft"
  Constant/1 -> Bus Creator5/1  "PwrMechLoss"
  Demux/3 -> Bus Creator6/3  "PwrAxl2"
  DriveshftTrq/1 -> Transferred Power/1
  Bus Creator7/1 -> Power Accounting Bus Creator/3
  Demux/2 -> Bus Creator6/2  "PwrAxl1"
  Demux/1 -> Bus Creator6/1  "PwrDriveshft"
  Speed/1 -> Transferred Power/2
  Vector Concatenate/1 -> Demux/1
  Constant1/1 -> Bus Creator5/2  "PwrDampLoss"
  Constant2/1 -> Bus Creator7/1  "PwrStoredShft"

== system EV6_LUT_FourWheel_EV6Battery77p4kWh_PowerCorrected/Vehicle Under Test1/Vehicle/Powertrain Supervisory Controller /Engine Torque Command/Accel Pedal to Traction Wheel Torque Request1 ==
  note: Convert Accelerator Pedal Position to Torque Command
      | using Motor Torque Speed Curve
  AccelPdl : Inport
  VehSpd_mph : Inport  Port=2
  2-D Lookup Table : Lookup_n-D  BreakpointsForDimension1=[0.0 0.1 0.2 0.3 0.4 0.5 0.6 0.7 0.8 0.9 1.0]  BreakpointsForDimension2=[0 10 20 30 40 50 60 70 80 90 100]  Table=|  InternalRulePriority=Speed  RndMeth=Simplest
      | [0,   0,   0,   0,   0,   0,   0,   0,   0,   0,   0;
      |     50,  36, 13,  10,   8,   5,   3,   2,   1,   0,   0;
      |    107,  75,  65,  60,  58,  45,  30,   18,   10,   4,   0;
      |    145, 108,  70,  63,  60,  52,  38,  25,  15,   6,   0;
      |    180, 168, 130,  95,  70,  52,  38,  27,  18,  10,   0;
      |    230, 220, 185, 145, 112,  85,  64,  47,  33,  21,   0;
      |    270, 258, 220, 178, 142, 112,  86,  65,  48,  34,  22;
      |    305, 295, 255, 212, 172, 138, 108,  83,  62,  45,  30;
      |    335, 325, 285, 240, 198, 160, 127,  98,  74,  54,  38;
      |    350, 345, 305, 258, 214, 174, 139, 108,  82,  60,  46; 360, 360, 325, 275, 228, 190, 158, 132, 108,  84,  60]
      settings: InputPortMap=u0,u1
  Max Motor Torque : Subsystem  Commented=on
  Product1 : Product
  Scope{,1..3} (4 alike) : Scope
  TrqCmd : Outport  VectorParamsAs1DForOutWhenUnconnected=off
  wires:
  VehSpd_mph/1 -> 2-D Lookup Table/2, Scope3/1  "TractionLUT_SpeedInput_mph"
  AccelPdl/1 -> 2-D Lookup Table/1, Scope/1  "TractionLUT_AccelInput"
  2-D Lookup Table/1 -> Scope1/1, TrqCmd/1  "TractionLUT_TorqueOutput_Nm"

== system EV6_LUT_FourWheel_EV6Battery77p4kWh_PowerCorrected/Vehicle Under Test1/Vehicle/Powertrain Supervisory Controller /Engine Torque Command/Battery Management System ==
  note: Behaviorial BMS System. Limits battery charge / discharge power based on SOC.
      |
      | Charge/Discharge Limits and curves can be adjusted if using a larger battery pack
      | or motor power is changed.
  SOC : Inport
  ChrgLmt : Lookup_n-D  NumberOfTableDimensions=1  BreakpointsForDimension1=BattChargeLimitSocBpts  Table=BattChargeLimitTbl  ExtrapMethod=Clip  UseLastTableValue=on  InternalRulePriority=Speed  RndMeth=Simplest
  DischrgLmt : Lookup_n-D  NumberOfTableDimensions=1  BreakpointsForDimension1=BattDischargeLimitSocBpts  Table=BattDischargeLimitTbl  ExtrapMethod=Clip  UseLastTableValue=on  InternalRulePriority=Speed  RndMeth=Simplest
  MaxChrg : Constant  Value=BattChargeLimitMaxPwr
  MaxDischrg : Constant  Value=BattDischargeMaxPwr
  Product : Product
  Product1 : Product
  BattPwrDischrgLmt : Outport  VectorParamsAs1DForOutWhenUnconnected=off
  BattPwrChrgLmt : Outport  Port=2  VectorParamsAs1DForOutWhenUnconnected=off
  wires:
  SOC/1 -> DischrgLmt/1, ChrgLmt/1
  MaxChrg/1 -> Product1/2
  MaxDischrg/1 -> Product/2
  Product/1 -> BattPwrDischrgLmt/1
  Product1/1 -> BattPwrChrgLmt/1
  ChrgLmt/1 -> Product1/1
  DischrgLmt/1 -> Product/1
